simulink model "afe_dqctrl_inv_psm"  (R2026a)
settings: Solver=ode23t  StopTime=simlength  FixedStep=tc  MaxStep=glb_time.tc  RelTol=1e-4
values from neighbouring files (symbols this model uses):
  afe_ctrl = ctrl_afe_setup(glb_time.ts_afe, grid_emu.omega_grid_nom)    [init_model.m]
  afe_pwm_phase_shift_mod1 = 0    [init_model.m]
  CTRPIFF_CLIP_RELEASE = 0.001    [init_model.m]
  filters = setup_global_filters(glb_time.ts_afe, glb_time.ts_inv, glb_time.ts_dab, glb_time.tc)    [init_model.m]
  glb_time = timing_setup(fpwm_afe, trgo_afe, fpwm_inv, trgo_inv, fpwm_single_phase_inv, trgo_single_phase_inv, fpwm_dab, trgo_dab,      fpwm_psfbc, trgo_psfbc, fpwm_isop_rail, trgo_isop_rail, fpwm_cllc, trgo_cllc, t_measure, tc_factor, tc_decimation, delay_pwm, dead_time_afe,      dead_time_inv, dead_time_single_phase_inv, dead_time_dab, dead_time_psfbc, dead_time_isop_rail, dead_time_cllc)    [init_model.m]
  grid_emu = grid_three_phase_emulator('Dyn11', delta_star, grid_nominal_power, application_voltage, us1, us2, fgrid,                  eq_grid_inductance, eq_grid_resistance, eta, ucc, i1m, p_iron, n1, n2, core_area, core_length, mur,                  up_xi_pu_ref, up_eta_pu_ref, un_xi_pu_ref, un_eta_pu_ref)    [init_model.m]
  heatsink = liquid_cooled_plate_2kw_setup(weight, no_weight, cp_al, heat_capacity_hs, thermal_conductivity_al,      Rth_switch_HA, Rth_mosfet_HA, Rth_diode_HA, Tambient, DThs_init)    [init_model.m]
  inv_pwm_phase_shift_mod1 = 0    [init_model.m]
  ki_align = 18    [init_model.m]
  kp_align = 0.25    [init_model.m]
  lim_down_align = -0.05    [init_model.m]
  lim_up_align = 0.05    [init_model.m]
  omega_m_sim = psm.omega_m_bez    [init_model.m]
  psm = psm_calculus()    [init_model.m]
  psm_ctrl = ctrl_pmsm_setup(glb_time.ts_inv, psm.omega_bez, u_psm_scale, psm.Jm_norm)    [init_model.m]
  simlength = 1.75    [init_model.m]
  Tambient = 40    [init_model.m]
  time_gain_afe_module_1 = 1.0002    [init_model.m]
  time_gain_inv_module_2 = 1.001    [init_model.m]
  time_start_motor_control = 0.25    [init_model.m]
  torque_overload_factor = 1.15    [init_model.m]
  u_cm_comp_mod1 = 0    [init_model.m]
  u_psm_scale_ekf = sqrt(3)/2 * 2/3 * hwdata.inv.udc_nom/psm.ubez    [init_model.m]
undefined symbols (not defined in the file or in its folder): hwdata, igbt, magnitude, omega_m_bez, rpm_base, torque_base
libraries: fl_lib x99, nesl_utility x96, igbt_simple_lib x12, single_phase_transformer_lib x3, threephase_inductor_lib x2, dclink_for_two_levels x2, three_phase_pwm_modulator x2, cstblocks_lti x2, discrete_time_low_pass_filter x1, lithium_ion_battery x1, three_phase_voltage_with_frt_emulator x1, simple_flexible_shaft x1
(part 5 of 9)

== system afe_dqctrl_inv_psm/inv_dq_mod1/INV_control/inverter_control/current_ctrl/current_ctrl ==
  iq_ref : Inport
  udc_pu : Inport  Port=2
  MTPA _mod1 : Subsystem
  Sqrt : Sqrt
  Square : Math  Operator=square
  Square1 : Math  Operator=square
  Sum : Sum  Inputs=|++
  dq_pi_with_vector_antiwindup mod1 : Subsystem
  id_ref _mod1 : Subsystem
      settings: PortSchema="{\"entries\":[{\"content\":{\"sides\":[{\"content\":{},\"type\":\"ConnectorPlacement.EquallySpacedRectSide\",\"uuid\":\"42af5d69-f0eb-42c6-9e03-28c1d0757323\"},{\"content\":{\"connectorIds\":[\"Out1\"],\"side\":\"RIGHT\"},\"type\":\"ConnectorPlacement.EquallySpacedRectSide\",\"uuid\":\"dd68a9f9-d15f-4e57-9d9e-130889a7b90c\"},{\"content\":{\"connectorIds\":[\"In1\"],\"side\":\"TOP\"},\"type\":\"ConnectorPlacement.EquallySpacedRectSide\",\"uuid\":\"68c797a2-8439-4b8d-8368-b7485adf0676\"}]},\"type\":\"ConnectorPlacement.EquallySpacedConnector\",\"uuid\":\"693c5f1c-0580-4626-8f13-b27865dfb3ac\"}],\"packageUris\":[\"http://schema.mathworks.com/mf0/Connector/R2020b\"],\"version\":\"1.0\"}"
  idref/id mod1 : Scope  NumInputPorts=2
      settings: ActiveDisplayYMinimum=-0.6792366431007606  ActiveDisplayYMaximum=0.075577635851628425
  iqref/iq mod1 : Scope  NumInputPorts=2
      settings: ActiveDisplayYMinimum=-2.4850184275737042  ActiveDisplayYMaximum=0.33436168402982208  DataLoggingVariableName=ScopeData2
  output voltage transformation : Subsystem
  tag scope: id_pu_ref_mod1=scoped, iq_pu_ref_mod1=scoped, u_mot_pu_mod1=scoped, ud_pu_mod1=scoped, uq_pu_mod1=scoped
  wires:
  [iq_pu_mod1] -> iqref/iq mod1/2, dq_pi_with_vector_antiwindup mod1/4(iq)  "iq"
  [id_pu_mod1] -> idref/id mod1/2, dq_pi_with_vector_antiwindup mod1/2(id)  "id"
  MTPA _mod1/1(Id_ref_mtpa) -> id_ref _mod1/1(id_mtpa), [id_pu_ref_mod1]  "id_ref"
  iq_ref/1 -> MTPA _mod1/1(iq_ref), iqref/iq mod1/1, dq_pi_with_vector_antiwindup mod1/3(iq_ref), [iq_pu_ref_mod1]  "iq_ref"
  dq_pi_with_vector_antiwindup mod1/1(ctrl_d_u) -> [ud_pu_mod1], Square1/1
  dq_pi_with_vector_antiwindup mod1/2(ctrl_q_u) -> [uq_pu_mod1], Square/1
  Square/1 -> Sum/1
  Sum/1 -> Sqrt/1
  Square1/1 -> Sum/2
  Sqrt/1 -> [u_mot_pu_mod1]
  id_ref _mod1/1(id_ref) -> idref/id mod1/1, dq_pi_with_vector_antiwindup mod1/1(id_ref)
  udc_pu/1 -> dq_pi_with_vector_antiwindup mod1/5(udc_pu)

== system afe_dqctrl_inv_psm/inv_dq_mod1/INV_control/inverter_control/current_ctrl/current_transformation ==
  Demux : Demux  Outputs=3
  alphabeta2dq : MATLAB Function  TreatAsAtomicUnit=on
  uvw2alphabeta : MATLAB Function  TreatAsAtomicUnit=on
  tag scope: ialpha_pu_mod1=scoped, ibeta_pu_mod1=scoped, id_pu_mod1=scoped, iq_pu_mod1=scoped
  wires:
  alphabeta2dq/2(q) -> [iq_pu_mod1]  "iq_pu"
  alphabeta2dq/1(d) -> [id_pu_mod1]  "id_pu"
  uvw2alphabeta/2(beta) -> alphabeta2dq/2(beta), [ibeta_pu_mod1]  "ibeta_pu"
  uvw2alphabeta/1(alpha) -> [ialpha_pu_mod1], alphabeta2dq/1(alpha)  "ialpha_pu"
  [motor_phase_ctrl_mod1] -> alphabeta2dq/3(gamma)
  Demux/3 -> uvw2alphabeta/3(w)  "iw"
  Demux/2 -> uvw2alphabeta/2(v)  "iv"
  Demux/1 -> uvw2alphabeta/1(u)  "iu"
  [isd_uvw_inv_mod1] -> Demux/1

== system afe_dqctrl_inv_psm/inv_dq_mod1/INV_control/inverter_control/encoder-sensorless-switch/double_integrator_observer ==
  phase_psm : Inport
  Dead Zone : DeadZone  LowerValue=-0.01  UpperValue=0.01
  Gain : Gain  Gain=psm_ctrl.di_obs.komega
  Gain1 : Gain  Gain=psm_ctrl.di_obs.ktheta
  Gain2 : Gain  Gain=psm_ctrl.omega_base
  Gain3 : Gain  Gain=1/psm_ctrl.omega_base
  Gain4 : Gain  Gain=glb_time.ts_inv
  Gain5 : Gain  Gain=glb_time.ts_inv
  Gain6 : Gain  Gain=glb_time.ts_inv
  Sum : Sum  Inputs=-+|
  Sum1 : Sum  Inputs=|++
  Sum2 : Sum  Inputs=|++
  Sum8 : Sum  Inputs=++|
  Unit Delay1 : UnitDelay  InitialCondition=pi  SampleTime=-1
  Unit Delay2 : UnitDelay  SampleTime=-1
  bounder1 : MATLAB Function  TreatAsAtomicUnit=on
  bounder2 : MATLAB Function  TreatAsAtomicUnit=on
  phase_psm_hat : Outport  VectorParamsAs1DForOutWhenUnconnected=off
  omega_pu_psm_hat : Outport  Port=2  VectorParamsAs1DForOutWhenUnconnected=off
  wires:
  Gain1/1 -> Gain6/1
  phase_psm/1 -> Sum/2
  Sum8/1 -> Unit Delay1/1
  Unit Delay1/1 -> bounder2/1(u)
  Sum1/1 -> Unit Delay2/1
  Gain/1 -> Gain4/1
  Unit Delay2/1 -> omega_pu_psm_hat/1, Sum1/2, Gain5/1
  Sum2/1 -> Sum8/2
  bounder2/1(y) -> Sum2/2, phase_psm_hat/1, Sum/1  "phase_hat"
  bounder1/1(y) -> Gain1/1, Gain/1
  Gain2/1 -> Sum8/1
  Gain3/1 -> Sum1/1
  Gain5/1 -> Gain2/1
  Sum/1 -> bounder1/1(u)
  Gain4/1 -> Gain3/1
  Gain6/1 -> Sum2/1

== system afe_dqctrl_inv_psm/inv_dq_mod1/INV_control/inverter_control/is inv quantizzation and one step delay/is inv quantizzation and one step delay ==
  is_u_pu : Inport
  is_v_pu : Inport  Port=2
  is_w_pu : Inport  Port=3
  Gain3 : Gain  Gain=-1
  Gain4 : Gain  Gain=-1
  Gain5 : Gain  Gain=-1
  Quantizer : Quantizer  QuantizationInterval=adc_quantization
  Quantizer1 : Quantizer  QuantizationInterval=adc_quantization
  Quantizer2 : Quantizer  QuantizationInterval=adc_quantization
  Unit Delay : UnitDelay  SampleTime=-1
  Unit Delay1 : UnitDelay  SampleTime=-1
  Unit Delay2 : UnitDelay  SampleTime=-1
  Zero-Order Hold : ZeroOrderHold  SampleTime=-1
  Zero-Order Hold1 : ZeroOrderHold  SampleTime=-1
  Zero-Order Hold2 : ZeroOrderHold  SampleTime=-1
  isd_u_pu : Outport
  isd_v_pu : Outport  Port=2
  isd_w_pu : Outport  Port=3
  wires:
  Unit Delay/1 -> Gain3/1
  Unit Delay1/1 -> Gain4/1
  Unit Delay2/1 -> Gain5/1
  Quantizer/1 -> Unit Delay/1
  Quantizer1/1 -> Unit Delay1/1
  Quantizer2/1 -> Unit Delay2/1
  is_u_pu/1 -> Zero-Order Hold/1
  is_v_pu/1 -> Zero-Order Hold1/1
  is_w_pu/1 -> Zero-Order Hold2/1
  Gain3/1 -> isd_u_pu/1
  Gain4/1 -> isd_v_pu/1
  Gain5/1 -> isd_w_pu/1
  Zero-Order Hold/1 -> Quantizer/1
  Zero-Order Hold1/1 -> Quantizer1/1
  Zero-Order Hold2/1 -> Quantizer2/1

== system afe_dqctrl_inv_psm/inv_dq_mod1/INV_control/inverter_control/omega_pu/flt ==
  input : Inport
  Gain3 : Gain  Gain=filters.inv.omega_flt_g1_10Hz
  Gain6 : Gain  Gain=filters.inv.omega_flt_g0_10Hz
  Sum : Sum  Inputs=|++
  Unit Delay1 : UnitDelay  SampleTime=-1
  output : Outport  VectorParamsAs1DForOutWhenUnconnected=off
  wires:
  Gain6/1 -> Sum/1
  input/1 -> Gain6/1
  Unit Delay1/1 -> Gain3/1
  Gain3/1 -> Sum/2
  Sum/1 -> Unit Delay1/1, output/1

== system afe_dqctrl_inv_psm/inv_dq_mod1/INV_control/inverter_control/phase_compensation_1/alignment_ctrl ==
  local_time : Inport
  master_time : Inport  Port=2
  Constant : Constant  Value=0
  Gain : Gain  Gain=-1
  Sum : Sum  Inputs=|+-
  pi : Subsystem  mask{kp=kp_align, ki=ki_align, lim_up=lim_up_align, lim_down=lim_down_align}
      mask prompts: ki "ki*ts"
      mask Display:
      | disp('pi()');
      | port_label('input', 1, 'u_ref');
      | port_label('input', 2, 'u');
      | port_label('output', 1, 'y');
  dp : Outport
  wires:
  master_time/1 -> Sum/1
  Sum/1 -> Gain/1
  Constant/1 -> pi/1(u_ref)
  local_time/1 -> Sum/2
  Gain/1 -> pi/2(u)
  pi/1(y) -> dp/1

== system afe_dqctrl_inv_psm/inv_dq_mod1/INV_control/inverter_control/speed_reference_generator/flt ==
  input : Inport
  Gain3 : Gain  Gain=filters.inv.g1_1Hz
  Gain6 : Gain  Gain=filters.inv.g0_1Hz
  Sum : Sum  Inputs=|++
  Unit Delay1 : UnitDelay  SampleTime=-1
  output : Outport  VectorParamsAs1DForOutWhenUnconnected=off
  wires:
  Gain6/1 -> Sum/1
  input/1 -> Gain6/1
  Unit Delay1/1 -> Gain3/1
  Gain3/1 -> Sum/2
  Sum/1 -> Unit Delay1/1, output/1

== system afe_dqctrl_inv_psm/inv_dq_mod1/inverter/inverter/sv_pwm/modulator1 ==
  u : Inport
  v : Inport  Port=2
  w : Inport  Port=3
  phase : Inport  Port=4
  Bus Creator : BusCreator  Inputs=3
  Three phase two level PWM generator with global TRGO : three_phase_pwm_modulator/Three phase two level PWM generator with global TRGO  f=glb_time.fPWM_INV  m_up=0.98  m_low=0.02  dead_time=glb_time.dead_time_INV  pos_cmd_gate=15  neg_cmd_gate=-10  polarity=1  tc=glb_time.tc  double_sampling=1
      link override gate commands/Bus Selector: OutputSignals=du(t)
      link override gate commands/Bus Selector1: OutputSignals=dv(t)
      link override gate commands/Bus Selector2: OutputSignals=dw(t)
  gate_cmds : Outport
  tag scope: TRGO_inv_module_1=global
  wires:
  [time_inv_module_1] -> Three phase two level PWM generator with global TRGO/1
  Bus Creator/1 -> Three phase two level PWM generator with global TRGO/3
  Three phase two level PWM generator with global TRGO/1 -> [TRGO_inv_module_1]
  u/1 -> Bus Creator/1
  v/1 -> Bus Creator/2
  w/1 -> Bus Creator/3
  phase/1 -> Three phase two level PWM generator with global TRGO/2
  Three phase two level PWM generator with global TRGO/2 -> gate_cmds/1

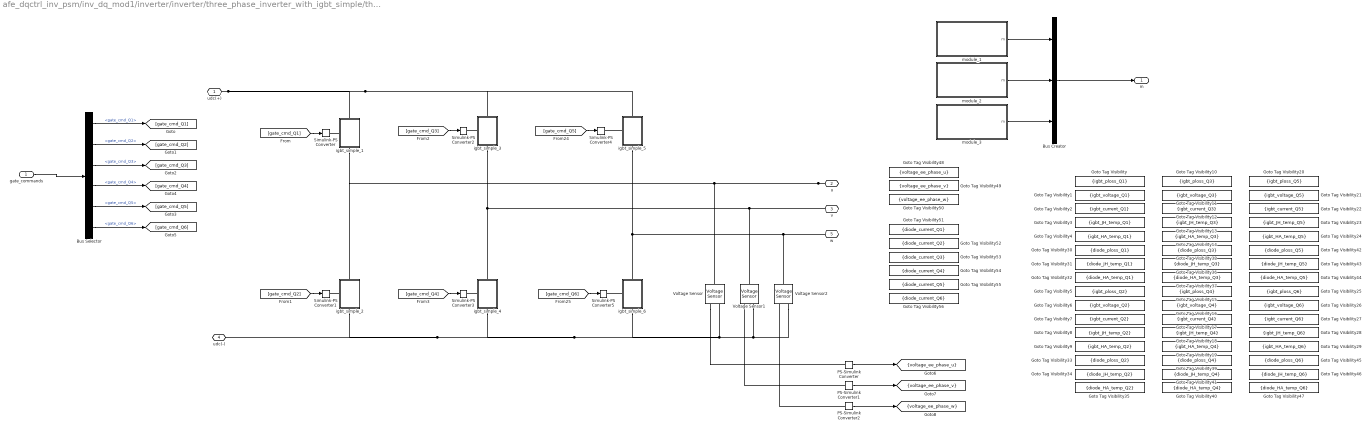
== system afe_dqctrl_inv_psm/inv_dq_mod1/inverter/inverter/three_phase_inverter_with_igbt_simple/three_phase_inverter_with_igbt_simple ==
  gate_commands : Inport
  Bus Creator : BusCreator  Inputs=3
  Bus Selector : BusSelector  OutputSignals=gate_cmd_Q1,gate_cmd_Q2,gate_cmd_Q3,gate_cmd_Q4,gate_cmd_Q5,gate_cmd_Q6
  Goto Tag Visibility : GotoTagVisibility  GotoTag=igbt_ploss_Q1
  Goto Tag Visibility1 : GotoTagVisibility  GotoTag=igbt_voltage_Q1
  Goto Tag Visibility10 : GotoTagVisibility  GotoTag=igbt_ploss_Q3
  Goto Tag Visibility11 : GotoTagVisibility  GotoTag=igbt_voltage_Q3
  Goto Tag Visibility12 : GotoTagVisibility  GotoTag=igbt_current_Q3
  Goto Tag Visibility13 : GotoTagVisibility  GotoTag=igbt_JH_temp_Q3
  Goto Tag Visibility14 : GotoTagVisibility  GotoTag=igbt_HA_temp_Q3
  Goto Tag Visibility15 : GotoTagVisibility  GotoTag=igbt_ploss_Q4
  Goto Tag Visibility16 : GotoTagVisibility  GotoTag=igbt_voltage_Q4
  Goto Tag Visibility17 : GotoTagVisibility  GotoTag=igbt_current_Q4
  Goto Tag Visibility18 : GotoTagVisibility  GotoTag=igbt_JH_temp_Q4
  Goto Tag Visibility19 : GotoTagVisibility  GotoTag=igbt_HA_temp_Q4
  Goto Tag Visibility2 : GotoTagVisibility  GotoTag=igbt_current_Q1
  Goto Tag Visibility20 : GotoTagVisibility  GotoTag=igbt_ploss_Q5
  Goto Tag Visibility21 : GotoTagVisibility  GotoTag=igbt_voltage_Q5
  Goto Tag Visibility22 : GotoTagVisibility  GotoTag=igbt_current_Q5
  Goto Tag Visibility23 : GotoTagVisibility  GotoTag=igbt_JH_temp_Q5
  Goto Tag Visibility24 : GotoTagVisibility  GotoTag=igbt_HA_temp_Q5
  Goto Tag Visibility25 : GotoTagVisibility  GotoTag=igbt_ploss_Q6
  Goto Tag Visibility26 : GotoTagVisibility  GotoTag=igbt_voltage_Q6
  Goto Tag Visibility27 : GotoTagVisibility  GotoTag=igbt_current_Q6
  Goto Tag Visibility28 : GotoTagVisibility  GotoTag=igbt_JH_temp_Q6
  Goto Tag Visibility29 : GotoTagVisibility  GotoTag=igbt_HA_temp_Q6
  Goto Tag Visibility3 : GotoTagVisibility  GotoTag=igbt_JH_temp_Q1
  Goto Tag Visibility30 : GotoTagVisibility  GotoTag=diode_ploss_Q1
  Goto Tag Visibility31 : GotoTagVisibility  GotoTag=diode_JH_temp_Q1
  Goto Tag Visibility32 : GotoTagVisibility  GotoTag=diode_HA_temp_Q1
  Goto Tag Visibility33 : GotoTagVisibility  GotoTag=diode_ploss_Q2
  Goto Tag Visibility34 : GotoTagVisibility  GotoTag=diode_JH_temp_Q2
  Goto Tag Visibility35 : GotoTagVisibility  GotoTag=diode_HA_temp_Q2
  Goto Tag Visibility36 : GotoTagVisibility  GotoTag=diode_JH_temp_Q3
  Goto Tag Visibility37 : GotoTagVisibility  GotoTag=diode_HA_temp_Q3
  Goto Tag Visibility38 : GotoTagVisibility  GotoTag=diode_ploss_Q3
  Goto Tag Visibility39 : GotoTagVisibility  GotoTag=diode_ploss_Q4
  Goto Tag Visibility4 : GotoTagVisibility  GotoTag=igbt_HA_temp_Q1
  Goto Tag Visibility40 : GotoTagVisibility  GotoTag=diode_HA_temp_Q4
  Goto Tag Visibility41 : GotoTagVisibility  GotoTag=diode_JH_temp_Q4
  Goto Tag Visibility42 : GotoTagVisibility  GotoTag=diode_ploss_Q5
  Goto Tag Visibility43 : GotoTagVisibility  GotoTag=diode_JH_temp_Q5
  Goto Tag Visibility44 : GotoTagVisibility  GotoTag=diode_HA_temp_Q5
  Goto Tag Visibility45 : GotoTagVisibility  GotoTag=diode_ploss_Q6
  Goto Tag Visibility46 : GotoTagVisibility  GotoTag=diode_JH_temp_Q6
  Goto Tag Visibility47 : GotoTagVisibility  GotoTag=diode_HA_temp_Q6
  Goto Tag Visibility48 : GotoTagVisibility  GotoTag=voltage_ee_phase_u
  Goto Tag Visibility49 : GotoTagVisibility  GotoTag=voltage_ee_phase_v
  Goto Tag Visibility5 : GotoTagVisibility  GotoTag=igbt_ploss_Q2
  Goto Tag Visibility50 : GotoTagVisibility  GotoTag=voltage_ee_phase_w
  Goto Tag Visibility51 : GotoTagVisibility  GotoTag=diode_current_Q1
  Goto Tag Visibility52 : GotoTagVisibility  GotoTag=diode_current_Q2
  Goto Tag Visibility53 : GotoTagVisibility  GotoTag=diode_current_Q3
  Goto Tag Visibility54 : GotoTagVisibility  GotoTag=diode_current_Q4
  Goto Tag Visibility55 : GotoTagVisibility  GotoTag=diode_current_Q5
  Goto Tag Visibility56 : GotoTagVisibility  GotoTag=diode_current_Q6
  Goto Tag Visibility6 : GotoTagVisibility  GotoTag=igbt_voltage_Q2
  Goto Tag Visibility7 : GotoTagVisibility  GotoTag=igbt_current_Q2
  Goto Tag Visibility8 : GotoTagVisibility  GotoTag=igbt_JH_temp_Q2
  Goto Tag Visibility9 : GotoTagVisibility  GotoTag=igbt_HA_temp_Q2
  PS-Simulink Converter : nesl_utility/PS-Simulink Converter  PhysicalDomain=network_engine_domain  SubClassName=ps_output  LeftPortType=input  RightPortType=output  PseudoPeriodic=off  Frequencies=[]  VectorFormat=1-D array  Unit=V  AffineConversion=off
  PS-Simulink Converter1 : nesl_utility/PS-Simulink Converter  PhysicalDomain=network_engine_domain  SubClassName=ps_output  LeftPortType=input  RightPortType=output  PseudoPeriodic=off  Frequencies=[]  VectorFormat=1-D array  Unit=V  AffineConversion=off
  PS-Simulink Converter2 : nesl_utility/PS-Simulink Converter  PhysicalDomain=network_engine_domain  SubClassName=ps_output  LeftPortType=input  RightPortType=output  PseudoPeriodic=off  Frequencies=[]  VectorFormat=1-D array  Unit=V  AffineConversion=off
  Simulink-PS Converter{,1..5} (6 alike) : nesl_utility/Simulink-PS Converter  PhysicalDomain=network_engine_domain  SubClassName=ps_input  LeftPortType=input  RightPortType=output  PseudoPeriodic=off  Frequencies=[]  NoiseDistribution=none  NoiseParameters=[]  Unit=V  AffineConversion=off  FilteringAndDerivatives=provide  SimscapeFilterOrder=1  InputFilterTimeConstant=0.001  UdotUserProvided=0
  Voltage Sensor : fl_lib/Electrical/Electrical Sensors/Voltage Sensor
  Voltage Sensor1 : fl_lib/Electrical/Electrical Sensors/Voltage Sensor
  Voltage Sensor2 : fl_lib/Electrical/Electrical Sensors/Voltage Sensor
  igbt_simple_1 : Subsystem
      settings: PortSchema="{\"entries\":[{\"content\":{\"sides\":[{\"content\":{\"connectorIds\":[\"LConn1\"]},\"type\":\"ConnectorPlacement.EquallySpacedRectSide\",\"uuid\":\"9277da8d-d460-43e6-8478-dd662f15d226\"},{\"content\":{\"connectorIds\":[],\"side\":\"RIGHT\"},\"type\":\"ConnectorPlacement.EquallySpacedRectSide\",\"uuid\":\"a7ece396-f1d9-4f4f-a05b-db1fc65d6e1d\"},{\"content\":{\"connectorIds\":[\"LConn2\"],\"side\":\"TOP\"},\"type\":\"ConnectorPlacement.EquallySpacedRectSide\",\"uuid\":\"fdd70777-e9cf-4317-afb6-cae87f75d5b0\"},{\"content\":{\"connectorIds\":[\"RConn1\"],\"side\":\"BOTTOM\"},\"type\":\"ConnectorPlacement.EquallySpacedRectSide\",\"uuid\":\"2353ed68-b1a1-4775-9ca9-31e268d5443b\"}]},\"type\":\"ConnectorPlacement.EquallySpacedConnector\",\"uuid\":\"d5479f4c-4e65-4791-adcb-73df11f88590\"}],\"packageUris\":[\"http://schema.mathworks.com/mf0/Connector/R2020b\"],\"version\":\"1.0\"}"
  igbt_simple_2 : Subsystem
      settings: PortSchema="{\"entries\":[{\"content\":{\"sides\":[{\"content\":{\"connectorIds\":[\"LConn1\"]},\"type\":\"ConnectorPlacement.EquallySpacedRectSide\",\"uuid\":\"9277da8d-d460-43e6-8478-dd662f15d226\"},{\"content\":{\"connectorIds\":[],\"side\":\"RIGHT\"},\"type\":\"ConnectorPlacement.EquallySpacedRectSide\",\"uuid\":\"a7ece396-f1d9-4f4f-a05b-db1fc65d6e1d\"},{\"content\":{\"connectorIds\":[\"LConn2\"],\"side\":\"TOP\"},\"type\":\"ConnectorPlacement.EquallySpacedRectSide\",\"uuid\":\"fdd70777-e9cf-4317-afb6-cae87f75d5b0\"},{\"content\":{\"connectorIds\":[\"RConn1\"],\"side\":\"BOTTOM\"},\"type\":\"ConnectorPlacement.EquallySpacedRectSide\",\"uuid\":\"2353ed68-b1a1-4775-9ca9-31e268d5443b\"}]},\"type\":\"ConnectorPlacement.EquallySpacedConnector\",\"uuid\":\"d5479f4c-4e65-4791-adcb-73df11f88590\"}],\"packageUris\":[\"http://schema.mathworks.com/mf0/Connector/R2020b\"],\"version\":\"1.0\"}"
  igbt_simple_3 : Subsystem
      settings: PortSchema="{\"entries\":[{\"content\":{\"sides\":[{\"content\":{\"connectorIds\":[\"LConn1\"]},\"type\":\"ConnectorPlacement.EquallySpacedRectSide\",\"uuid\":\"9277da8d-d460-43e6-8478-dd662f15d226\"},{\"content\":{\"connectorIds\":[],\"side\":\"RIGHT\"},\"type\":\"ConnectorPlacement.EquallySpacedRectSide\",\"uuid\":\"a7ece396-f1d9-4f4f-a05b-db1fc65d6e1d\"},{\"content\":{\"connectorIds\":[\"LConn2\"],\"side\":\"TOP\"},\"type\":\"ConnectorPlacement.EquallySpacedRectSide\",\"uuid\":\"fdd70777-e9cf-4317-afb6-cae87f75d5b0\"},{\"content\":{\"connectorIds\":[\"RConn1\"],\"side\":\"BOTTOM\"},\"type\":\"ConnectorPlacement.EquallySpacedRectSide\",\"uuid\":\"2353ed68-b1a1-4775-9ca9-31e268d5443b\"}]},\"type\":\"ConnectorPlacement.EquallySpacedConnector\",\"uuid\":\"d5479f4c-4e65-4791-adcb-73df11f88590\"}],\"packageUris\":[\"http://schema.mathworks.com/mf0/Connector/R2020b\"],\"version\":\"1.0\"}"
  igbt_simple_4 : Subsystem
      settings: PortSchema="{\"entries\":[{\"content\":{\"sides\":[{\"content\":{\"connectorIds\":[\"LConn1\"]},\"type\":\"ConnectorPlacement.EquallySpacedRectSide\",\"uuid\":\"9277da8d-d460-43e6-8478-dd662f15d226\"},{\"content\":{\"connectorIds\":[],\"side\":\"RIGHT\"},\"type\":\"ConnectorPlacement.EquallySpacedRectSide\",\"uuid\":\"a7ece396-f1d9-4f4f-a05b-db1fc65d6e1d\"},{\"content\":{\"connectorIds\":[\"LConn2\"],\"side\":\"TOP\"},\"type\":\"ConnectorPlacement.EquallySpacedRectSide\",\"uuid\":\"fdd70777-e9cf-4317-afb6-cae87f75d5b0\"},{\"content\":{\"connectorIds\":[\"RConn1\"],\"side\":\"BOTTOM\"},\"type\":\"ConnectorPlacement.EquallySpacedRectSide\",\"uuid\":\"2353ed68-b1a1-4775-9ca9-31e268d5443b\"}]},\"type\":\"ConnectorPlacement.EquallySpacedConnector\",\"uuid\":\"d5479f4c-4e65-4791-adcb-73df11f88590\"}],\"packageUris\":[\"http://schema.mathworks.com/mf0/Connector/R2020b\"],\"version\":\"1.0\"}"
  igbt_simple_5 : Subsystem
      settings: PortSchema="{\"entries\":[{\"content\":{\"sides\":[{\"content\":{\"connectorIds\":[\"LConn1\"]},\"type\":\"ConnectorPlacement.EquallySpacedRectSide\",\"uuid\":\"9277da8d-d460-43e6-8478-dd662f15d226\"},{\"content\":{\"connectorIds\":[],\"side\":\"RIGHT\"},\"type\":\"ConnectorPlacement.EquallySpacedRectSide\",\"uuid\":\"a7ece396-f1d9-4f4f-a05b-db1fc65d6e1d\"},{\"content\":{\"connectorIds\":[\"LConn2\"],\"side\":\"TOP\"},\"type\":\"ConnectorPlacement.EquallySpacedRectSide\",\"uuid\":\"fdd70777-e9cf-4317-afb6-cae87f75d5b0\"},{\"content\":{\"connectorIds\":[\"RConn1\"],\"side\":\"BOTTOM\"},\"type\":\"ConnectorPlacement.EquallySpacedRectSide\",\"uuid\":\"2353ed68-b1a1-4775-9ca9-31e268d5443b\"}]},\"type\":\"ConnectorPlacement.EquallySpacedConnector\",\"uuid\":\"d5479f4c-4e65-4791-adcb-73df11f88590\"}],\"packageUris\":[\"http://schema.mathworks.com/mf0/Connector/R2020b\"],\"version\":\"1.0\"}"
  igbt_simple_6 : Subsystem
      settings: PortSchema="{\"entries\":[{\"content\":{\"sides\":[{\"content\":{\"connectorIds\":[\"LConn1\"]},\"type\":\"ConnectorPlacement.EquallySpacedRectSide\",\"uuid\":\"9277da8d-d460-43e6-8478-dd662f15d226\"},{\"content\":{\"connectorIds\":[],\"side\":\"RIGHT\"},\"type\":\"ConnectorPlacement.EquallySpacedRectSide\",\"uuid\":\"a7ece396-f1d9-4f4f-a05b-db1fc65d6e1d\"},{\"content\":{\"connectorIds\":[\"LConn2\"],\"side\":\"TOP\"},\"type\":\"ConnectorPlacement.EquallySpacedRectSide\",\"uuid\":\"fdd70777-e9cf-4317-afb6-cae87f75d5b0\"},{\"content\":{\"connectorIds\":[\"RConn1\"],\"side\":\"BOTTOM\"},\"type\":\"ConnectorPlacement.EquallySpacedRectSide\",\"uuid\":\"2353ed68-b1a1-4775-9ca9-31e268d5443b\"}]},\"type\":\"ConnectorPlacement.EquallySpacedConnector\",\"uuid\":\"d5479f4c-4e65-4791-adcb-73df11f88590\"}],\"packageUris\":[\"http://schema.mathworks.com/mf0/Connector/R2020b\"],\"version\":\"1.0\"}"
  module_1 : Subsystem
  module_2 : Subsystem
  module_3 : Subsystem
  udc(+) : PMIOPort  Side=Left
  u : PMIOPort  Port=2  Side=Right
  v : PMIOPort  Port=3  Side=Right
  udc(-) : PMIOPort  Port=4  Side=Left
  w : PMIOPort  Port=5  Side=Right
  m : Outport
  tag scope: voltage_ee_phase_u=scoped, voltage_ee_phase_v=scoped, voltage_ee_phase_w=scoped
  wires:
  module_3/1(m) -> Bus Creator/3
  module_1/1(m) -> Bus Creator/1
  Bus Creator/1 -> m/1
  module_2/1(m) -> Bus Creator/2
  PS-Simulink Converter2/1 -> [voltage_ee_phase_w]
  PS-Simulink Converter1/1 -> [voltage_ee_phase_v]
  PS-Simulink Converter/1 -> [voltage_ee_phase_u]
  [gate_cmd_Q6] -> Simulink-PS Converter5/1
  [gate_cmd_Q5] -> Simulink-PS Converter4/1
  [gate_cmd_Q3] -> Simulink-PS Converter2/1
  [gate_cmd_Q4] -> Simulink-PS Converter3/1
  [gate_cmd_Q2] -> Simulink-PS Converter1/1
  [gate_cmd_Q1] -> Simulink-PS Converter/1
  gate_commands/1 -> Bus Selector/1
  Bus Selector/6 -> [gate_cmd_Q6]  "<gate_cmd_Q6>"
  Bus Selector/5 -> [gate_cmd_Q5]  "<gate_cmd_Q5>"
  Bus Selector/4 -> [gate_cmd_Q4]  "<gate_cmd_Q4>"
  Bus Selector/3 -> [gate_cmd_Q3]  "<gate_cmd_Q3>"
  Bus Selector/2 -> [gate_cmd_Q2]  "<gate_cmd_Q2>"
  Bus Selector/1 -> [gate_cmd_Q1]  "<gate_cmd_Q1>"
  connections:
  PS-Simulink Converter2/LConn1 -- Voltage Sensor2/RConn1
  PS-Simulink Converter1/LConn1 -- Voltage Sensor1/RConn1
  Voltage Sensor/RConn1 -- PS-Simulink Converter/LConn1
  w/RConn1 -- Voltage Sensor2/LConn1 -- igbt_simple_6/LConn2 -- igbt_simple_5/RConn1
  v/RConn1 -- Voltage Sensor1/LConn1 -- igbt_simple_4/LConn2 -- igbt_simple_3/RConn1
  Voltage Sensor1/RConn2 -- Voltage Sensor2/RConn2 -- Voltage Sensor/RConn2 -- igbt_simple_6/RConn1 -- igbt_simple_4/RConn1 -- igbt_simple_2/RConn1 -- udc(-)/RConn1
  igbt_simple_6/LConn1 -- Simulink-PS Converter5/RConn1
  igbt_simple_5/LConn1 -- Simulink-PS Converter4/RConn1
  igbt_simple_4/LConn1 -- Simulink-PS Converter3/RConn1
  igbt_simple_3/LConn1 -- Simulink-PS Converter2/RConn1
  igbt_simple_2/LConn1 -- Simulink-PS Converter1/RConn1
  igbt_simple_1/LConn1 -- Simulink-PS Converter/RConn1
  udc(+)/RConn1 -- igbt_simple_1/LConn2 -- igbt_simple_5/LConn2 -- igbt_simple_3/LConn2
  u/RConn1 -- Voltage Sensor/LConn1 -- igbt_simple_2/LConn2 -- igbt_simple_1/RConn1

== system afe_dqctrl_inv_psm/afe_dq_mod1/AFE_control/afe_control/acquisitions/ig afe quantizzation and one step delay/ig afe quantizzation and one step delay ==
  ig_u_pu : Inport
  ig_v_pu : Inport  Port=2
  ig_w_pu : Inport  Port=3
  Gain4 : Gain  Gain=-1
  Gain5 : Gain  Gain=-1
  Gain6 : Gain  Gain=-1
  Quantizer1 : Quantizer  QuantizationInterval=adc_quantization
  Quantizer2 : Quantizer  QuantizationInterval=adc_quantization
  Quantizer4 : Quantizer  QuantizationInterval=adc_quantization
  Unit Delay : UnitDelay  SampleTime=-1
  Unit Delay1 : UnitDelay  SampleTime=-1
  Unit Delay2 : UnitDelay  SampleTime=-1
  Zero-Order Hold : ZeroOrderHold  SampleTime=-1
  Zero-Order Hold1 : ZeroOrderHold  SampleTime=-1
  Zero-Order Hold2 : ZeroOrderHold  SampleTime=-1
  igd_u_pu : Outport
  igd_v_pu : Outport  Port=2
  igd_w_pu : Outport  Port=3
  wires:
  Quantizer1/1 -> Unit Delay1/1
  Quantizer4/1 -> Unit Delay/1
  Quantizer2/1 -> Unit Delay2/1
  ig_u_pu/1 -> Zero-Order Hold/1
  ig_v_pu/1 -> Zero-Order Hold1/1
  ig_w_pu/1 -> Zero-Order Hold2/1
  Unit Delay/1 -> Gain4/1
  Unit Delay1/1 -> Gain5/1
  Unit Delay2/1 -> Gain6/1
  Gain4/1 -> igd_u_pu/1
  Gain5/1 -> igd_v_pu/1
  Gain6/1 -> igd_w_pu/1
  Zero-Order Hold/1 -> Quantizer4/1
  Zero-Order Hold1/1 -> Quantizer1/1
  Zero-Order Hold2/1 -> Quantizer2/1

== system afe_dqctrl_inv_psm/afe_dq_mod1/AFE_control/afe_control/acquisitions/is afe quantizzation and one step delay/is afe quantizzation and one step delay ==
  is_u_pu : Inport
  is_v_pu : Inport  Port=2
  is_w_pu : Inport  Port=3
  Quantizer : Quantizer  QuantizationInterval=adc_quantization
  Quantizer1 : Quantizer  QuantizationInterval=adc_quantization
  Quantizer2 : Quantizer  QuantizationInterval=adc_quantization
  Unit Delay : UnitDelay  SampleTime=-1
  Unit Delay1 : UnitDelay  SampleTime=-1
  Unit Delay2 : UnitDelay  SampleTime=-1
  Zero-Order Hold : ZeroOrderHold  SampleTime=-1
  Zero-Order Hold1 : ZeroOrderHold  SampleTime=-1
  Zero-Order Hold2 : ZeroOrderHold  SampleTime=-1
  isd_u_pu : Outport
  isd_v_pu : Outport  Port=2
  isd_w_pu : Outport  Port=3
  wires:
  Unit Delay/1 -> isd_u_pu/1
  Unit Delay1/1 -> isd_v_pu/1
  Unit Delay2/1 -> isd_w_pu/1
  Quantizer/1 -> Unit Delay/1
  Quantizer1/1 -> Unit Delay1/1
  Quantizer2/1 -> Unit Delay2/1
  is_u_pu/1 -> Zero-Order Hold/1
  is_v_pu/1 -> Zero-Order Hold1/1
  is_w_pu/1 -> Zero-Order Hold2/1
  Zero-Order Hold/1 -> Quantizer/1
  Zero-Order Hold1/1 -> Quantizer1/1
  Zero-Order Hold2/1 -> Quantizer2/1

== system afe_dqctrl_inv_psm/afe_dq_mod1/AFE_control/afe_control/acquisitions/phase_compensation_1/alignment_eval_afe1 ==
  local_time : Inport
  master_time : Inport  Port=2
  Constant : Constant  Value=0
  Gain : Gain  Gain=-1
  Sum : Sum  Inputs=|+-
  pi : Subsystem  mask{kp=kp_align, ki=ki_align*glb_time.ts_afe, lim_up=lim_up_align, lim_down=lim_down_align}
      mask prompts: ki "ki*ts"
      mask Display:
      | disp('pi()');
      | port_label('input', 1, 'u_ref');
      | port_label('input', 2, 'u');
      | port_label('output', 1, 'y');
  dp : Outport
  wires:
  master_time/1 -> Sum/1
  Sum/1 -> Gain/1
  Constant/1 -> pi/1(u_ref)
  local_time/1 -> Sum/2
  Gain/1 -> pi/2(u)
  pi/1(y) -> dp/1

== system afe_dqctrl_inv_psm/afe_dq_mod1/AFE_control/afe_control/acquisitions/ug afe quantizzation and one step delay/ug afe quantizzation and one step delay ==
  ug_u_pu : Inport
  ug_v_pu : Inport  Port=2
  ug_w_pu : Inport  Port=3
  Quantizer1 : Quantizer  QuantizationInterval=adc_quantization
  Quantizer2 : Quantizer  QuantizationInterval=adc_quantization
  Quantizer4 : Quantizer  QuantizationInterval=adc_quantization
  Unit Delay : UnitDelay  SampleTime=-1
  Unit Delay1 : UnitDelay  SampleTime=-1
  Unit Delay2 : UnitDelay  SampleTime=-1
  Zero-Order Hold : ZeroOrderHold  SampleTime=-1
  Zero-Order Hold1 : ZeroOrderHold  SampleTime=-1
  Zero-Order Hold2 : ZeroOrderHold  SampleTime=-1
  ugd_u_pu : Outport
  ugd_v_pu : Outport  Port=2
  ugd_w_pu : Outport  Port=3
  wires:
  Unit Delay/1 -> ugd_u_pu/1
  Unit Delay1/1 -> ugd_v_pu/1
  Unit Delay2/1 -> ugd_w_pu/1
  Quantizer4/1 -> Unit Delay/1
  Quantizer1/1 -> Unit Delay1/1
  Quantizer2/1 -> Unit Delay2/1
  ug_w_pu/1 -> Zero-Order Hold2/1
  ug_v_pu/1 -> Zero-Order Hold1/1
  ug_u_pu/1 -> Zero-Order Hold/1
  Zero-Order Hold/1 -> Quantizer4/1
  Zero-Order Hold1/1 -> Quantizer1/1
  Zero-Order Hold2/1 -> Quantizer2/1

== system afe_dqctrl_inv_psm/afe_dq_mod1/AFE_control/afe_control/current_ctrl/dq_vector_pi/bounder1 ==
  md : Inport
  m_1 : Inport  Port=2
  m : Inport  Port=3
  Constant : Constant
  Constant1 : Constant  Value=0
  Divide : Product
  Switch : Switch  Threshold=1  SaturateOnIntegerOverflow=off  InputSameDT=off
  Switch1 : Switch  Threshold=1  SaturateOnIntegerOverflow=off  InputSameDT=off
  md_sat : Outport  VectorParamsAs1DForOutWhenUnconnected=off
  clip : Outport  Port=2  VectorParamsAs1DForOutWhenUnconnected=off
  wires:
  md/1 -> Switch1/3, Divide/2
  m_1/1 -> Divide/1
  Divide/1 -> Switch1/1
  Switch1/1 -> md_sat/1
  Switch/1 -> clip/1
  m/1 -> Switch/2, Switch1/2
  Constant/1 -> Switch/1
  Constant1/1 -> Switch/3

== system afe_dqctrl_inv_psm/afe_dq_mod1/AFE_control/afe_control/current_ctrl/dq_vector_pi/bounder2 ==
  m : Inport
  m_1 : Inport  Port=2
  mq : Inport  Port=3
  Constant : Constant
  Constant1 : Constant  Value=0
  Divide : Product
  Switch : Switch  Threshold=1  SaturateOnIntegerOverflow=off  InputSameDT=off
  Switch1 : Switch  Threshold=1  SaturateOnIntegerOverflow=off  InputSameDT=off
  mq_sat : Outport  VectorParamsAs1DForOutWhenUnconnected=off
  clip : Outport  Port=2  VectorParamsAs1DForOutWhenUnconnected=off
  wires:
  Constant1/1 -> Switch/3
  Constant/1 -> Switch/1
  m/1 -> Switch1/2, Switch/2
  Switch/1 -> clip/1
  Switch1/1 -> mq_sat/1
  Divide/1 -> Switch1/1
  m_1/1 -> Divide/1
  mq/1 -> Divide/2, Switch1/3

== system afe_dqctrl_inv_psm/afe_dq_mod1/AFE_control/afe_control/current_ctrl/dq_vector_pi/pi_d ==
  id_tilde : Inport
  clip : Inport  Port=2
  1/Ti : Gain  Gain=psm_ctrl.kp_i  SaturateOnIntegerOverflow=on  OutDataTypeStr=Inherit: Same as input  ParamDataTypeStr=Inherit: Same as input
  Constant : Constant  Value=0
  Sum2 : Sum  Inputs=+-  SaturateOnIntegerOverflow=on
  Sum4 : Sum  SaturateOnIntegerOverflow=on
  Sum5 : Sum  SaturateOnIntegerOverflow=on
  Switch1 : Switch  Threshold=0.5  SaturateOnIntegerOverflow=off  InputSameDT=off
  Switch2 : Switch  Threshold=0.5  SaturateOnIntegerOverflow=off  InputSameDT=off
  Unit Delay1 : UnitDelay  SampleTime=-1
  Unit Delay2 : UnitDelay  SampleTime=-1
  kp1 : Gain  Gain=CTRPIFF_CLIP_RELEASE*glb_time.ts_inv  SaturateOnIntegerOverflow=on  OutDataTypeStr=Inherit: Same as input  ParamDataTypeStr=Inherit: Same as input
  kp2 : Gain  Gain=psm_ctrl.ki_i*glb_time.ts_inv  SaturateOnIntegerOverflow=on  OutDataTypeStr=Inherit: Same as input  ParamDataTypeStr=Inherit: Same as input
  ud_out : Outport  VectorParamsAs1DForOutWhenUnconnected=off
  wires:
  id_tilde/1 -> kp2/1, 1/Ti/1
  Sum5/1 -> ud_out/1
  Switch1/1 -> Unit Delay2/1
  Sum4/1 -> Sum5/2, Switch1/3
  kp1/1 -> Sum2/2
  Sum2/1 -> Switch1/1
  Unit Delay2/1 -> Sum4/2, kp1/1, Sum2/1
  1/Ti/1 -> Sum5/1
  Switch2/1 -> Sum4/1
  kp2/1 -> Switch2/3
  clip/1 -> Unit Delay1/1
  [clip] -> Switch2/2
  [clip] -> Switch1/2
  Constant/1 -> Switch2/1
  Unit Delay1/1 -> [clip]

== system afe_dqctrl_inv_psm/afe_dq_mod1/AFE_control/afe_control/current_ctrl/dq_vector_pi/pi_q ==
  iq_tilde : Inport
  clip : Inport  Port=2
  1/Ti : Gain  Gain=psm_ctrl.kp_i  SaturateOnIntegerOverflow=on  OutDataTypeStr=Inherit: Same as input  ParamDataTypeStr=Inherit: Same as input
  Constant : Constant  Value=0
  Sum2 : Sum  Inputs=+-  SaturateOnIntegerOverflow=on
  Sum4 : Sum  SaturateOnIntegerOverflow=on
  Sum5 : Sum  SaturateOnIntegerOverflow=on
  Switch1 : Switch  Threshold=0.5  SaturateOnIntegerOverflow=off  InputSameDT=off
  Switch2 : Switch  Threshold=0.5  SaturateOnIntegerOverflow=off  InputSameDT=off
  Unit Delay1 : UnitDelay  SampleTime=-1
  Unit Delay2 : UnitDelay  SampleTime=-1
  kp1 : Gain  Gain=CTRPIFF_CLIP_RELEASE*glb_time.ts_inv  SaturateOnIntegerOverflow=on  OutDataTypeStr=Inherit: Same as input  ParamDataTypeStr=Inherit: Same as input
  kp2 : Gain  Gain=psm_ctrl.ki_i*glb_time.ts_inv  SaturateOnIntegerOverflow=on  OutDataTypeStr=Inherit: Same as input  ParamDataTypeStr=Inherit: Same as input
  Vqs_out : Outport  VectorParamsAs1DForOutWhenUnconnected=off
  wires:
  Constant/1 -> Switch2/1
  [clip] -> Switch1/2
  [clip] -> Switch2/2
  clip/1 -> Unit Delay1/1
  kp2/1 -> Switch2/3
  Switch2/1 -> Sum4/1
  1/Ti/1 -> Sum5/1
  Unit Delay2/1 -> Sum2/1, kp1/1, Sum4/2
  Sum2/1 -> Switch1/1
  kp1/1 -> Sum2/2
  Sum4/1 -> Sum5/2, Switch1/3
  Switch1/1 -> Unit Delay2/1
  iq_tilde/1 -> 1/Ti/1, kp2/1
  Unit Delay1/1 -> [clip]
  Sum5/1 -> Vqs_out/1

== system afe_dqctrl_inv_psm/afe_dq_mod1/AFE_control/afe_control/current_ctrl/dq_vector_pi/switch ==
  clip 1 : Inport
  clip 2 : Inport  Port=2
  Constant4 : Constant
  Constant5 : Constant  Value=0
  Sum1 : Sum  SaturateOnIntegerOverflow=on
  Switch : Switch  Threshold=0.5  SaturateOnIntegerOverflow=off  InputSameDT=off
  clip : Outport  VectorParamsAs1DForOutWhenUnconnected=off
  wires:
  Constant5/1 -> Switch/3
  Switch/1 -> clip/1
  Constant4/1 -> Switch/1
  Sum1/1 -> Switch/2
  clip 1/1 -> Sum1/1
  clip 2/1 -> Sum1/2

== system afe_dqctrl_inv_psm/afe_dq_mod1/AFE_control/afe_control/current_ctrl/dq_vector_pi/vector lenght ==
  md : Inport
  mq : Inport  Port=2
  Math Function : Math  Operator=magnitude^2  SignedPower=on
  Math Function1 : Math  Operator=magnitude^2  SignedPower=on
  Math Function2 : Math  Operator=reciprocal  SignedPower=on
  Sqrt : Sqrt
  Sum5 : Sum  SaturateOnIntegerOverflow=on
  m_1 : Outport  VectorParamsAs1DForOutWhenUnconnected=off
  m : Outport  Port=2  VectorParamsAs1DForOutWhenUnconnected=off
  wires:
  Sqrt/1 -> m/1, Math Function2/1
  mq/1 -> Math Function1/1
  Math Function1/1 -> Sum5/2
  Math Function/1 -> Sum5/1
  Sum5/1 -> Sqrt/1
  Math Function2/1 -> m_1/1
  md/1 -> Math Function/1

== system afe_dqctrl_inv_psm/afe_dq_mod1/AFE_control/afe_control/current_ctrl/zero_current_ctrl/iz ==
  Demux : Demux  Outputs=3
  Gain : Gain  Gain=1/3
  Sum : Sum  Inputs=+++
  iz : Outport
  wires:
  Sum/1 -> Gain/1
  Demux/1 -> Sum/1  "is_a"
  [isd_abc_pu] -> Demux/1
  Demux/3 -> Sum/3  "is_c"
  Demux/2 -> Sum/2  "is_b"
  Gain/1 -> iz/1

== system afe_dqctrl_inv_psm/afe_dq_mod1/AFE_control/afe_control/current_ctrl/zero_current_ctrl/zero_sequence_current_ctrl ==
  iz : Inport
  1/Ti : Gain  Gain=afe_ctrl.kp_is_z  SaturateOnIntegerOverflow=on  OutDataTypeStr=Inherit: Same as input  ParamDataTypeStr=Inherit: Same as input
  Constant1 : Constant  Value=0
  Gain : Gain
  Saturation : Saturate  UpperLimit=1  LowerLimit=-1
  Sum1 : Sum  Inputs=+++  SaturateOnIntegerOverflow=on
  Sum2 : Sum  Inputs=-+  SaturateOnIntegerOverflow=on
  Sum3 : Sum  Inputs=-+  SaturateOnIntegerOverflow=on
  Unit Delay4 : UnitDelay  SampleTime=-1
  iz_tracking : Scope  NumInputPorts=3
      settings: ActiveDisplayYMinimum=-1  ActiveDisplayYMaximum=1  DataLoggingVariableName=ScopeData8
  kp : Gain  Gain=afe_ctrl.ki_is_z*glb_time.ts_afe  SaturateOnIntegerOverflow=on  OutDataTypeStr=Inherit: Same as input  ParamDataTypeStr=Inherit: Same as input
  ugamma_afe : Outport
  tag scope: iz_ctrl_out=scoped, iz_pu=scoped, iz_pu_ref=scoped
  wires:
  1/Ti/1 -> Sum1/1, Sum3/1
  kp/1 -> Sum1/2
  Sum3/1 -> Unit Delay4/1
  Unit Delay4/1 -> Sum1/3
  Constant1/1 -> [iz_pu_ref], iz_tracking/1, Sum2/2  "iz_pu_ref"
  iz/1 -> [iz_pu], iz_tracking/2, Sum2/1  "iz_pu"
  Sum2/1 -> kp/1, 1/Ti/1
  Sum1/1 -> Saturation/1
  Saturation/1 -> Gain/1, [iz_ctrl_out], iz_tracking/3, Sum3/2  "iz_ctrl_out"
  Gain/1 -> ugamma_afe/1

== system afe_dqctrl_inv_psm/afe_dq_mod1/AFE_control/afe_control/grid_voltage_phase_lock_loops/FHT-PLL/pll_stageA ==
  gamma_grid : Inport
  ug_abc_pu : Inport  Port=2
  Demux : Demux  Outputs=3
  Math Function : Math  Operator=magnitude^2  SignedPower=on
  Math Function1 : Math  Operator=magnitude^2  SignedPower=on
  Reciprocal Sqrt : Sqrt  Operator=rSqrt
  Saturation : Saturate  UpperLimit=inf  LowerLimit=0.02
  Sum : Sum  Inputs=|++
  filter_and_transformation : Subsystem
  sequences : Subsystem
  u_grid_xi : Outport  VectorParamsAs1DForOutWhenUnconnected=off
  u_grid_eta : Outport  Port=2  VectorParamsAs1DForOutWhenUnconnected=off
  tag scope: Vgrid_unorm_fht=scoped
  wires:
  gamma_grid/1 -> sequences/3(phase_angle)
  sequences/2(u_grid_eta) -> u_grid_eta/1
  sequences/1(u_grid_xi) -> u_grid_xi/1
  ug_abc_pu/1 -> Demux/1
  Demux/1 -> filter_and_transformation/1(ug_a)
  Demux/2 -> filter_and_transformation/2(ug_b)
  Demux/3 -> filter_and_transformation/3(ug_c)
  filter_and_transformation/1(ug_alpha) -> Math Function/1, sequences/1(u_grid_alpha)
  filter_and_transformation/2(ug_beta) -> Math Function1/1, sequences/2(u_grid_beta)
  Math Function/1 -> Sum/1
  Math Function1/1 -> Sum/2
  Sum/1 -> Saturation/1
  Reciprocal Sqrt/1 -> [Vgrid_unorm_fht]
  Saturation/1 -> Reciprocal Sqrt/1

== system afe_dqctrl_inv_psm/afe_dq_mod1/AFE_control/afe_control/grid_voltage_phase_lock_loops/FHT-PLL/pll_stageB ==
  u_grid_pos_xi : Inport
  u_grid_pos_eta : Inport  Port=2
  Constant4 : Constant  Value=grid_emu.omega_grid_nom
  Gain : Gain  Gain=-1
  Product : Product  RndMeth=Zero
  Product1 : Product  RndMeth=Zero
  Product2 : Product  RndMeth=Zero
  Sum3 : Sum  SaturateOnIntegerOverflow=on
  Sum4 : Sum  SaturateOnIntegerOverflow=on
  Sum5 : Sum  Inputs=++|
  Terminator : Terminator
  Unit Delay1 : UnitDelay  SampleTime=-1
  Unit Delay2 : UnitDelay  SampleTime=-1
  Unit Delay4 : UnitDelay  SampleTime=-1
  bounder1 : MATLAB Function  TreatAsAtomicUnit=on
  double_integrator_observer : Subsystem
  kp : Gain  Gain=afe_ctrl.pll_i1_fht*glb_time.ts_afe  SaturateOnIntegerOverflow=on  OutDataTypeStr=Inherit: Same as input  ParamDataTypeStr=Inherit: Same as input
  kp1 : Gain  Gain=afe_ctrl.pll_p_fht  SaturateOnIntegerOverflow=on  OutDataTypeStr=Inherit: Same as input  ParamDataTypeStr=Inherit: Same as input
  kp2 : Gain  Gain=glb_time.ts_afe  SaturateOnIntegerOverflow=on  OutDataTypeStr=Inherit: Same as input  ParamDataTypeStr=Inherit: Same as input
  kp3 : Gain  Gain=1/grid_emu.omega_grid_nom  SaturateOnIntegerOverflow=on  OutDataTypeStr=Inherit: Same as input  ParamDataTypeStr=Inherit: Same as input
  gamma_grid_ddsrf_pll : Outport  VectorParamsAs1DForOutWhenUnconnected=off
  omega_grid_ddsrf_pll : Outport  Port=2  VectorParamsAs1DForOutWhenUnconnected=off
  wires:
  Gain/1 -> kp/1, kp1/1
  Product1/1 -> Gain/1
  kp3/1 -> omega_grid_ddsrf_pll/1
  Product/1 -> Terminator/1
  double_integrator_observer/1(omega_hat) -> kp3/1
  Unit Delay4/1 -> Sum3/2
  Sum4/1 -> bounder1/1(u)
  Unit Delay1/1 -> Sum4/2
  Sum3/1 -> Sum5/2, Unit Delay4/1  "i1"
  kp2/1 -> Sum4/1
  Constant4/1 -> Product2/2
  [Vgrid_unorm_fht] -> Product/2, Product1/2
  kp/1 -> Sum3/1
  Sum5/1 -> Product2/1
  bounder1/1(y) -> Unit Delay2/1, Unit Delay1/1
  u_grid_pos_xi/1 -> Product/1
  u_grid_pos_eta/1 -> Product1/1
  Product2/1 -> kp2/1
  kp1/1 -> Sum5/1
  Unit Delay2/1 -> double_integrator_observer/1(theta), gamma_grid_ddsrf_pll/1

== system afe_dqctrl_inv_psm/afe_dq_mod1/AFE_control/afe_control/grid_voltage_phase_lock_loops/FHT-PLL_simulink/pll_stageA ==
  gamma_grid : Inport
  ug_abc_pu : Inport  Port=2
  Demux : Demux  Outputs=3
  Math Function : Math  Operator=magnitude^2  SignedPower=on
  Math Function1 : Math  Operator=magnitude^2  SignedPower=on
  Reciprocal Sqrt : Sqrt  Operator=rSqrt
  Saturation : Saturate  UpperLimit=inf  LowerLimit=0.02
  Sum : Sum  Inputs=|++
  filter_and_transformation : Subsystem
  sequences : Subsystem
  u_grid_xi : Outport  VectorParamsAs1DForOutWhenUnconnected=off
  u_grid_eta : Outport  Port=2  VectorParamsAs1DForOutWhenUnconnected=off
  tag scope: Vgrid_unorm_fht_simulink=scoped
  wires:
  Saturation/1 -> Reciprocal Sqrt/1
  Reciprocal Sqrt/1 -> [Vgrid_unorm_fht_simulink]
  Sum/1 -> Saturation/1
  Math Function1/1 -> Sum/2
  Math Function/1 -> Sum/1
  filter_and_transformation/2(ug_beta) -> sequences/2(u_grid_beta), Math Function1/1
  filter_and_transformation/1(ug_alpha) -> sequences/1(u_grid_alpha), Math Function/1
  Demux/3 -> filter_and_transformation/3(ug_c)
  Demux/2 -> filter_and_transformation/2(ug_b)
  Demux/1 -> filter_and_transformation/1(ug_a)
  ug_abc_pu/1 -> Demux/1
  sequences/1(u_grid_xi) -> u_grid_xi/1
  sequences/2(u_grid_eta) -> u_grid_eta/1
  gamma_grid/1 -> sequences/3(phase_angle)

== system afe_dqctrl_inv_psm/afe_dq_mod1/AFE_control/afe_control/grid_voltage_phase_lock_loops/FHT-PLL_simulink/pll_stageB ==
  u_grid_pos_xi : Inport
  u_grid_pos_eta : Inport  Port=2
  Constant4 : Constant  Value=grid_emu.omega_grid_nom
  Gain : Gain  Gain=-1
  Product : Product  RndMeth=Zero
  Product1 : Product  RndMeth=Zero
  Product2 : Product  RndMeth=Zero
  Sum3 : Sum  SaturateOnIntegerOverflow=on
  Sum4 : Sum  SaturateOnIntegerOverflow=on
  Sum5 : Sum  Inputs=++|
  Terminator : Terminator
  Unit Delay1 : UnitDelay  SampleTime=-1
  Unit Delay2 : UnitDelay  SampleTime=-1
  Unit Delay4 : UnitDelay  SampleTime=-1
  bounder1 : MATLAB Function  TreatAsAtomicUnit=on
  double_integrator_observer : Subsystem
  kp : Gain  Gain=afe_ctrl.pll_i1_fht*glb_time.ts_afe  SaturateOnIntegerOverflow=on  OutDataTypeStr=Inherit: Same as input  ParamDataTypeStr=Inherit: Same as input
  kp1 : Gain  Gain=afe_ctrl.pll_p_fht  SaturateOnIntegerOverflow=on  OutDataTypeStr=Inherit: Same as input  ParamDataTypeStr=Inherit: Same as input
  kp2 : Gain  Gain=glb_time.ts_afe  SaturateOnIntegerOverflow=on  OutDataTypeStr=Inherit: Same as input  ParamDataTypeStr=Inherit: Same as input
  kp3 : Gain  Gain=1/grid_emu.omega_grid_nom  SaturateOnIntegerOverflow=on  OutDataTypeStr=Inherit: Same as input  ParamDataTypeStr=Inherit: Same as input
  gamma_grid_ddsrf_pll : Outport  VectorParamsAs1DForOutWhenUnconnected=off
  omega_grid_ddsrf_pll : Outport  Port=2  VectorParamsAs1DForOutWhenUnconnected=off
  wires:
  Unit Delay2/1 -> gamma_grid_ddsrf_pll/1, double_integrator_observer/1(theta)
  kp1/1 -> Sum5/1
  Product2/1 -> kp2/1
  u_grid_pos_eta/1 -> Product1/1
  u_grid_pos_xi/1 -> Product/1
  bounder1/1(y) -> Unit Delay1/1, Unit Delay2/1
  Sum5/1 -> Product2/1
  kp/1 -> Sum3/1
  [Vgrid_unorm_fht_simulink] -> Product1/2, Product/2
  Constant4/1 -> Product2/2
  kp2/1 -> Sum4/1
  Sum3/1 -> Unit Delay4/1, Sum5/2  "i1"
  Unit Delay1/1 -> Sum4/2
  Sum4/1 -> bounder1/1(u)
  Unit Delay4/1 -> Sum3/2
  double_integrator_observer/1(omega_hat) -> kp3/1
  Product/1 -> Terminator/1
  kp3/1 -> omega_grid_ddsrf_pll/1
  Product1/1 -> Gain/1
  Gain/1 -> kp1/1, kp/1

== system afe_dqctrl_inv_psm/afe_dq_mod1/AFE_control/afe_control/grid_voltage_phase_lock_loops/dq_pll/pll_stageA ==
  phase_grid : Inport
  ug_abc : Inport  Port=2
  Demux : Demux  Outputs=3
  Math Function : Math  Operator=magnitude^2  SignedPower=on
  Math Function1 : Math  Operator=magnitude^2  SignedPower=on
  Reciprocal Sqrt : Sqrt  Operator=rSqrt
  Saturation : Saturate  UpperLimit=inf  LowerLimit=0.02
  Sum : Sum  Inputs=|++
  mormalization_and_transformation : Subsystem
  sequences : Subsystem
  u_grid_pos_xi : Outport  VectorParamsAs1DForOutWhenUnconnected=off
  u_grid_pos_eta : Outport  Port=2  VectorParamsAs1DForOutWhenUnconnected=off
  tag scope: Vgrid_unorm_dqpll=scoped
  wires:
  ug_abc/1 -> Demux/1
  Demux/1 -> mormalization_and_transformation/1(ug_a)
  Demux/2 -> mormalization_and_transformation/2(ug_b)
  Demux/3 -> mormalization_and_transformation/3(ug_c)
  phase_grid/1 -> sequences/3(gamma_grid)
  sequences/1(u_grid_pos_xi) -> u_grid_pos_xi/1
  sequences/2(u_grid_pos_eta) -> u_grid_pos_eta/1
  Math Function1/1 -> Sum/2
  mormalization_and_transformation/1(ug_alpha) -> Math Function/1, sequences/1(u_grid_alpha)
  mormalization_and_transformation/2(ug_beta) -> Math Function1/1, sequences/2(u_grid_beta)
  Reciprocal Sqrt/1 -> [Vgrid_unorm_dqpll]
  Sum/1 -> Saturation/1
  Math Function/1 -> Sum/1
  Saturation/1 -> Reciprocal Sqrt/1

== system afe_dqctrl_inv_psm/afe_dq_mod1/AFE_control/afe_control/grid_voltage_phase_lock_loops/dq_pll/pll_stageB ==
  u_grid_pos_xi : Inport
  u_grid_pos_eta : Inport  Port=2
  -2<x<2 : Saturate  UpperLimit=2  LowerLimit=-2
  Constant4 : Constant  Value=grid_emu.omega_grid_nom
  Gain : Gain  Gain=1/grid_emu.omega_grid_nom
  Product1 : Product  RndMeth=Zero
  Product2 : Product  RndMeth=Zero
  Sum3 : Sum  SaturateOnIntegerOverflow=on
  Sum4 : Sum  SaturateOnIntegerOverflow=on
  Sum5 : Sum  Inputs=++|
  Terminator : Terminator
  Unit Delay1 : UnitDelay  SampleTime=-1
  Unit Delay2 : UnitDelay  SampleTime=-1
  Unit Delay4 : UnitDelay  SampleTime=-1
  bounder1 : MATLAB Function  TreatAsAtomicUnit=on
  double_integrator_observer : Subsystem
  kp : Gain  Gain=afe_ctrl.pll_i1*glb_time.ts_afe  SaturateOnIntegerOverflow=on  OutDataTypeStr=Inherit: Same as input  ParamDataTypeStr=Inherit: Same as input
  kp2 : Gain  Gain=glb_time.ts_afe  SaturateOnIntegerOverflow=on  OutDataTypeStr=Inherit: Same as input  ParamDataTypeStr=Inherit: Same as input
  scheduled-p-gain : Subsystem
      settings: PortSchema="{\"entries\":[{\"content\":{\"sides\":[{\"content\":{},\"type\":\"ConnectorPlacement.EquallySpacedRectSide\",\"uuid\":\"88e64df2-a299-4c1b-9bac-7a615cd04a00\"},{\"content\":{\"side\":\"RIGHT\"},\"type\":\"ConnectorPlacement.EquallySpacedRectSide\",\"uuid\":\"ef1d7318-b0e2-4e96-bf99-c42bb4ec5202\"},{\"content\":{\"connectorIds\":[\"In1\"],\"side\":\"TOP\"},\"type\":\"ConnectorPlacement.EquallySpacedRectSide\",\"uuid\":\"96582c59-f6c8-40f1-b3cf-394cc239c4b2\"},{\"content\":{\"connectorIds\":[\"Out1\"],\"side\":\"BOTTOM\"},\"type\":\"ConnectorPlacement.EquallySpacedRectSide\",\"uuid\":\"9ac5cd0d-958f-4b67-b4ea-90856a0aa038\"}]},\"type\":\"ConnectorPlacement.EquallySpacedConnector\",\"uuid\":\"ca37db80-6b94-4315-bd9c-66307567cd1f\"}],\"packageUris\":[\"http://schema.mathworks.com/mf0/Connector/R2020b\"],\"version\":\"1.0\"}"
  phase_grid_pll : Outport  VectorParamsAs1DForOutWhenUnconnected=off
  omega_grid_pu_pll : Outport  Port=2  VectorParamsAs1DForOutWhenUnconnected=off
  wires:
  Unit Delay4/1 -> Sum3/2
  Sum3/1 -> -2<x<2/1
  Sum4/1 -> bounder1/1(u)
  Unit Delay1/1 -> Sum4/2
  -2<x<2/1 -> Sum5/2, Unit Delay4/1  "i1"
  kp2/1 -> Sum4/1
  Constant4/1 -> Product2/2
  [Vgrid_unorm_dqpll] -> Product1/2
  kp/1 -> Sum3/1
  Sum5/1 -> Product2/1
  bounder1/1(y) -> Unit Delay1/1, Unit Delay2/1
  u_grid_pos_eta/1 -> Product1/1
  Product2/1 -> kp2/1
  Product1/1 -> scheduled-p-gain/1(In1), kp/1
  scheduled-p-gain/1(Out2) -> Sum5/1
  Unit Delay2/1 -> double_integrator_observer/1(phase), phase_grid_pll/1
  double_integrator_observer/1(omega_hat) -> Gain/1
  Gain/1 -> omega_grid_pu_pll/1
  u_grid_pos_xi/1 -> Terminator/1
